simulink model "ModeLogic_MVP_AI"  (R2026b)
settings: Solver=ode4  StopTime=90  FixedStep=0.005
settings Model: DataDictionary=QuadInterfaces_AI.sldd  Creator=JonathanTee  LastModifiedBy=JonathanTee

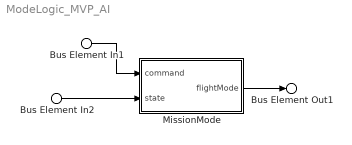
== system ModeLogic_MVP_AI ==
  Bus Element In1 : Inport  PortName=MissionCommand
  Bus Element In2 : Inport  Port=2  PortName=VehicleState
  MissionMode : MATLAB Function  TreatAsAtomicUnit=on
  Bus Element Out1 : Outport  PortName=FlightMode
  wires:
  MissionMode/1(flightMode) -> Bus Element Out1/1
  Bus Element In2/1 -> MissionMode/2(state)
  Bus Element In1/1 -> MissionMode/1(command)

== matlab function ModeLogic_MVP_AI/MissionMode ==
  settings: updateMethod=DISCRETE  sampleTime=MVP.SampleTime
  data: command input Bus: MissionCommand_IF; flightMode output Bus: FlightMode_IF; state input Bus: VehicleState_IF
function flightMode=modeLogic(command,state)
%#codegen
flightMode=stage02_mode_logic(command,state);
end
